simulink model "Project4_Sim"  (R2019a)
settings: Solver=ode4  StartTime=0.0  StopTime=tf  FixedStep=0.1  RelTol=1e-3
values from neighbouring files (symbols this model uses):
  yd = [50; 50; 0; 0; 0; 0]    [CW_Matrix.m]    (also in Controller.m = u(7:12); Project4_Main.m = [rho_f;drho_f]; Riccati.m = defaultReference)
undefined symbols (not defined in the file or in its folder): Controller, CW_Equation, Output
settings Model: Creator=Andrew  LastModifiedBy=Andrew

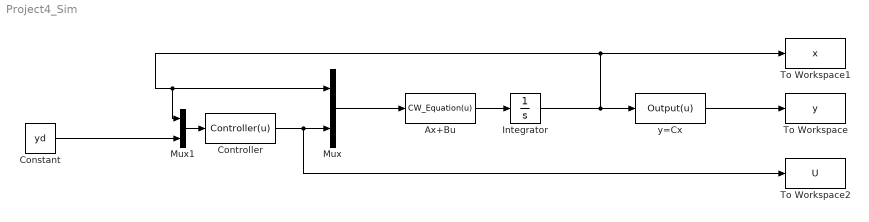
== system Project4_Sim ==
  Ax+Bu : MATLABFcn  MATLABFcn=CW_Equation(u)  OutputDimensions=6
  Constant : Constant  Value=yd
  "Controller " : MATLABFcn  MATLABFcn=Controller(u)
  Integrator : Integrator  InitialCondition=[100;200;20;1;-1;0.5]
  Mux : Mux  Inputs=[6;3]
  Mux1 : Mux  Inputs=[6;6]
  To Workspace : ToWorkspace  VariableName=y  SaveFormat=Timeseries  SampleTime=-1
  To Workspace1 : ToWorkspace  VariableName=x  SaveFormat=Timeseries  SampleTime=-1
  To Workspace2 : ToWorkspace  VariableName=U  SaveFormat=Timeseries  SampleTime=-1
  y=Cx : MATLABFcn  MATLABFcn=Output(u)
  wires:
  Ax+Bu/1 -> Integrator/1
  Integrator/1 -> To Workspace1/1, Mux1/1, Mux/1, y=Cx/1
  y=Cx/1 -> To Workspace/1
  Mux/1 -> Ax+Bu/1
  "Controller "/1 -> Mux/2, To Workspace2/1
  Mux1/1 -> "Controller "/1
  Constant/1 -> Mux1/2
